simulink model "EncoderSpeed"  (R2026b)
settings: Solver=VariableStepAuto
values from neighbouring files (symbols this model uses):
  Enc_DirSign = 1    [DCMotorParams.m]
  Spd_CalDivisor = Spd_RawAt100/Motor_NoLoadRpm    (= 1.20345454545)    [DCMotorParams.m]
  Spd_RpmPerCount = 60/(Enc_CPR_Output*Spd_WindowN*Ts)    (= 5.68181818182)    [DCMotorParams.m]
  Spd_WindowN = 5    [DCMotorParams.m]
  Ts = 0.01    [DCMotorParams.m]
libraries: arduinosensorlib x1
settings Model: Creator=bence  LastModifiedBy=bence

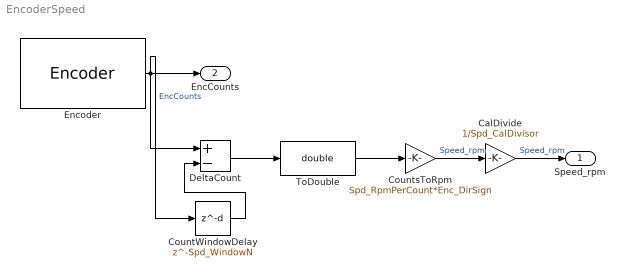
== system EncoderSpeed ==
  CalDivide : Gain  Gain=1/Spd_CalDivisor
  CountWindowDelay : Delay  DelayLength=Spd_WindowN  InitialCondition=0
  CountsToRpm : Gain  Gain=Spd_RpmPerCount*Enc_DirSign
  DeltaCount : Sum  Inputs=+-
  Encoder : arduinosensorlib/Encoder  InputA=Enc_PinA  InputB=Enc_PinB  Mode=No reset  SampleTime=Ts
  ToDouble : DataTypeConversion  OutDataTypeStr=double  SaturateOnIntegerOverflow=off  RndMeth=Floor
  Speed_rpm : Outport
  EncCounts : Outport  Port=2
  wires:
  CountsToRpm/1 -> CalDivide/1  "Speed_rpm"
  CalDivide/1 -> Speed_rpm/1  "Speed_rpm"
  ToDouble/1 -> CountsToRpm/1
  DeltaCount/1 -> ToDouble/1
  CountWindowDelay/1 -> DeltaCount/2
  Encoder/1 -> DeltaCount/1, CountWindowDelay/1, EncCounts/1  "EncCounts"
